simulink model "sf_fitness"  (R2025b)
settings: Solver=FixedStepAuto  StartTime=0.0  StopTime=inf  FixedStep=0.001  RelTol=1e-3  EnableMultiTasking=on
PreLoadFcn:
  | load sf_fitness_buses.mat;
StopFcn:
  | delete(app)
undefined symbols (not defined in the file or in its folder): ActivityType
CloseFcn:
  | clear app
  | clear FitnessDisplay
  | clear FitnessThresholds
  | clear FitnessVitals
settings Model: Creator=The MathWorks, Inc.  LastModifiedBy=The MathWorks, Inc.
settings SolverCC: AlgebraicLoopSolver=TrustRegion  IsAutoAppliedInSIP=on
settings DataIOCC: LimitDataPoints=on  SaveTime=off  ReturnWorkspaceOutputs=off
settings OptimizationCC: ReuseModelBlockBuffer=off  LifeSpan=inf
settings DebuggingCC: UnconnectedInputMsg=warning  UnconnectedOutputMsg=warning  UnconnectedLineMsg=warning  AllowSymbolicDim=off  PregeneratedLibrarySubsystemCodeDiagnostic=none  SFUnexpectedBacktrackingDiag=warning  SFNoUnconditionalDefaultTransitionDiag=warning  SFExecutionAtInitializationDiag=none  ArithmeticOperatorsInVariantConditions=warning
settings ModelReferenceCC: EnableRefExpFcnMdlSchedulingChecks=on  PropagateSignalLabelsOutOfModel=off
settings SFSimCC: SimUseLocalCustomCode=off  CustomCodeUndefinedFunction=UseInterfaceOnly
settings RTWCC: RTWUseLocalCustomCode=off  GPUComputeCapability=3.5  DLArmComputeVersion=19.05
settings CodeAppCC: StateflowObjectComments=on
settings GRTTargetCC: TargetLangStandard=C89/C90 (ANSI)
settings ConfigComp: CovMetricSettings=dw  CovSaveCumulativeToWorkspaceVar=on  CovSaveSingleToWorkspaceVar=on  CovExternalEMLEnable=off
settings SimscapeCC: SimscapeNormalizeSystem=off  SimscapeNominalValues={1, 'bar'; 1, 'cm^3/s'; 1, 'bar*kg/s'; 1, 'kJ/kg'; 1, 'kW'}

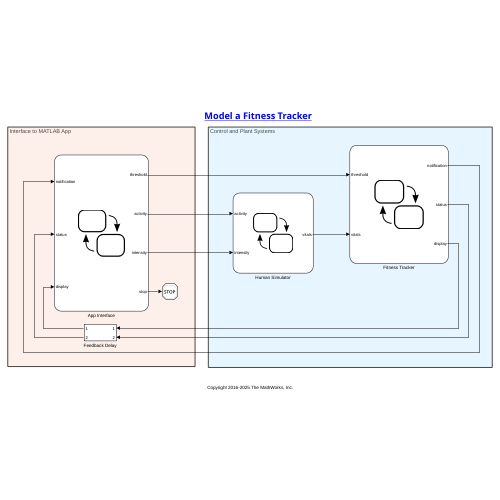
[thumbnail: Simulink's stored preview of the top-level diagram]
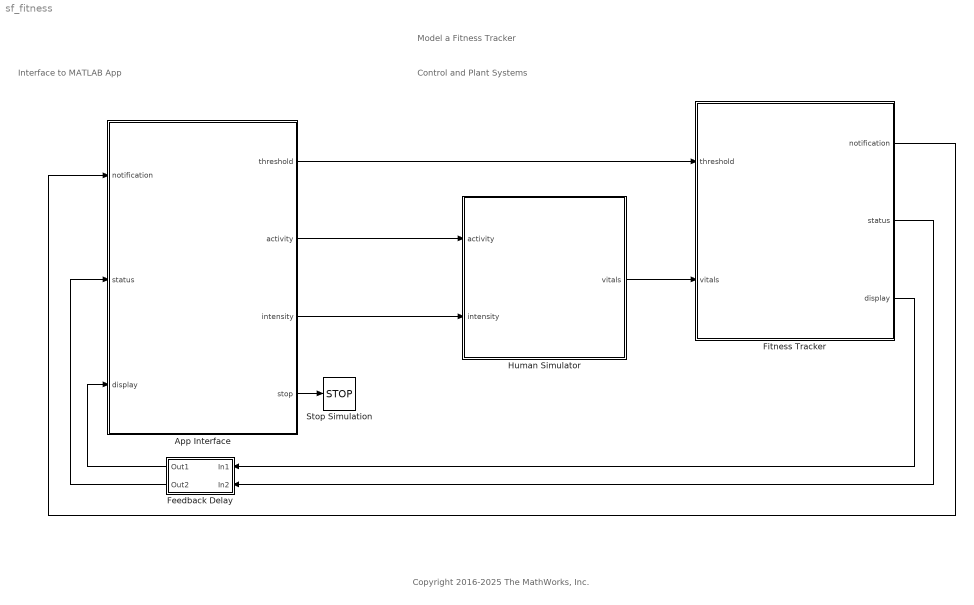
== system sf_fitness ==
  note: Control and Plant Systems
  note: Interface to MATLAB App
  note: Copyright 2016-2025 The MathWorks, Inc.
  note: Model a Fitness Tracker
  App Interface : Stateflow chart  TreatAsAtomicUnit=on
  Feedback Delay : Subsystem
  Fitness Tracker : Stateflow chart  TreatAsAtomicUnit=on
      settings: PortSchema="{\"entries\":[{\"content\":{\"sides\":[{\"content\":{\"connectorIds\":[\"In1\",\"In2\"]},\"type\":\"ConnectorPlacement.EquallySpacedRectSide\",\"uuid\":\"afd40bc3-205b-45f1-b484-c4f33cea0ca8\"},{\"content\":{\"connectorIds\":[\"Out1\",\"Out3\",\"Out2\"],\"side\":\"RIGHT\"},\"type\":\"ConnectorPlacement.EquallySpacedRectSide\",\"uuid\":\"d6f91233-35c5-46a8-af22-1c26ecf92787\"},{\"content\":{\"connectorIds\":[],\"side\":\"TOP\"},\"type\":\"ConnectorPlacement.EquallySpacedRectSide\",\"uuid\":\"b785bd09-019e-4ae9-a457-04601cbf60c7\"},{\"content\":{\"connectorIds\":[],\"side\":\"HIDDEN\"},\"type\":\"ConnectorPlacement.EquallySpacedRectSide\",\"uuid\":\"2c22bb70-70b2-4576-b4f3-3c6d9d9d65de\"}]},\"type\":\"ConnectorPlacement.EquallySpacedConnector\",\"uuid\":\"fb400832-b5be-41c1-a3a6-f64440305270\"}],\"packageUris\":[\"http://schema.mathworks.com/mf0/Connector/R2020b\"],\"version\":\"1.0\"}"
  Human Simulator : Stateflow chart  TreatAsAtomicUnit=on
  Stop Simulation : Stop
  wires:
  App Interface/4(stop) -> Stop Simulation/1
  App Interface/2(activity) -> Human Simulator/1(activity)
  App Interface/3(intensity) -> Human Simulator/2(intensity)
  Fitness Tracker/1(notification) -> App Interface/1(notification)
  Fitness Tracker/2(display) -> Feedback Delay/1(In1)
  Feedback Delay/2(Out2) -> App Interface/2(status)
  Feedback Delay/1(Out1) -> App Interface/3(display)
  App Interface/1(threshold) -> Fitness Tracker/1(threshold)
  Human Simulator/1(vitals) -> Fitness Tracker/2(vitals)
  Fitness Tracker/3(" status") -> Feedback Delay/2(In2)

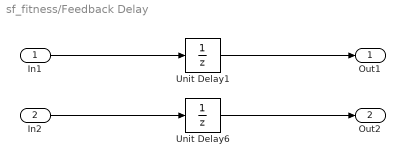
== system sf_fitness/Feedback Delay ==
  In1 : Inport
  In2 : Inport  Port=2
  Unit Delay1 : UnitDelay  SampleTime=-1  HasFrameUpgradeWarning=on
  Unit Delay6 : UnitDelay  InitialCondition=ActivityType.Rest  SampleTime=-1  HasFrameUpgradeWarning=on
  Out1 : Outport
  Out2 : Outport  Port=2
  wires:
  Unit Delay6/1 -> Out2/1
  In1/1 -> Unit Delay1/1
  Unit Delay1/1 -> Out1/1
  In2/1 -> Unit Delay6/1

== stateflow chart sf_fitness/Human Simulator ==
  note: Units for variables:
      | speed: number of steps per second
      | heart_rate: beats per minute
  state Simulator [parallel]
    en:
    vitals.heart_rate = 75;
    vitals.speed = 0;
    settings: executionOrder=1
    state Sim_Sleep
      en:
      oldhr = vitals.heart_rate;
      olds = vitals.speed;
      oldt = t;
      du:
      [vitals.heart_rate,vitals.speed] = sim_sleep(oldhr,olds,t-oldt);
    state Sim_Rest
      en:
      oldhr = vitals.heart_rate;
      olds = vitals.speed;
      oldt = t;
      du:
      [vitals.heart_rate,vitals.speed] = sim_rest(oldhr,olds,t-oldt);
    state Sim_Walk
      en:
      oldhr = vitals.heart_rate;
      olds = vitals.speed;
      oldt = t;
      du:
      [vitals.heart_rate,vitals.speed] = sim_walk(oldhr,olds,t-oldt);
    state Sim_Exercise
      en:
      oldhr = vitals.heart_rate;
      olds = vitals.speed;
      oldt = t;
      du:
      [vitals.heart_rate,vitals.speed] = sim_exercise(oldhr,olds,t-oldt,intensity);
    (default) -> (junction 353)
    (junction 353) -> (junction 257)
    (junction 257) -> Sim_Sleep [order 1] : [activity == ActivityType.Sleep]
    Sim_Sleep -> (junction 280)
    (junction 288) -> (junction 353)
    (junction 257) -> (junction 262) [order 2]
    (junction 280) -> (junction 281)
    (junction 262) -> Sim_Rest [order 1] : [activity == ActivityType.Rest]
    Sim_Rest -> (junction 281)
    (junction 262) -> (junction 264) [order 2]
    (junction 281) -> (junction 282)
    (junction 264) -> Sim_Walk [order 1] : [activity == ActivityType.Walk]
    Sim_Walk -> (junction 282)
    (junction 264) -> (junction 266) [order 2]
    (junction 282) -> (junction 286)
    (junction 266) -> Sim_Exercise : %[activity == ActivityType.Exercise]
    Sim_Exercise -> (junction 286)
    (junction 286) -> (junction 287)
    (junction 287) -> (junction 288) : [hasChanged(activity) || hasChanged(intensity)]
  state Step_Tracker [parallel]
    en: vitals.steps = 0;
    settings: executionOrder=2
    state Step
    (default) -> Step
    Step -> Step : after(1,sec){vitals.steps = vitals.steps + vitals.speed * 60;}
  data: oldHR function_input; oldS function_input; newTime function_input; heartRate function_output; Speed function_output; oldHR function_input; oldS function_input; newTime function_input; heartRate function_output; Speed function_output; oldHR function_input; oldS function_input; newTime function_input; heartRate function_output; Speed function_output; heartRate function_output; Speed function_output; oldHR function_input; oldS function_input; newTime function_input; Strength function_input; old function_input; target function_input; result function_output; t function_input; activity input Enum: ActivityType; intensity input; oldhr local; olds local; oldt local; vitals output Bus: FitnessVitals size=1
  function [heartRate, Speed] = sim_sleep(oldHR, oldS, newTime):
    | function [heartRate, Speed] = sim_sleep(oldHR, oldS, newTime)
    |    
    | target = 68;
    | 
    | % call transition function from oldHR to target
    | heartRate = transition(oldHR, target, newTime);
    | % update exercising speed
    | Speed = transition(oldS, 0, newTime);
    |     
    | end
  function [heartRate, Speed] = sim_rest(oldHR, oldS, newTime):
    | function [heartRate, Speed] = sim_rest(oldHR, oldS, newTime)
    |    
    | target = 75;
    | 
    | % call transition function from oldHR to target
    | heartRate = transition(oldHR, target, newTime);
    | % update exercising speed
    | Speed = transition(oldS, 0, newTime);
    |     
    | end
  function [heartRate, Speed] = sim_walk(oldHR, oldS, newTime):
    | function [heartRate, Speed] = sim_walk(oldHR, oldS, newTime)
    |    
    | target = 85;
    | 
    | % call transition function from oldHR to target
    | heartRate = transition(oldHR, target, newTime);
    | % update exercising speed
    | Speed = transition(oldS, 2, newTime);
    |     
    | end
  function [heartRate, Speed] = sim_exercise(oldHR, oldS, newTime, Strength):
    | function [heartRate, Speed] = sim_exercise(oldHR, oldS, newTime, Strength)
    | 
    | % strength is exercise level 1- 10
    | target = 85 + Strength * 8;
    | 
    | % call transition function from oldHR to target
    | heartRate = transition(oldHR, target, newTime);
    | % update exercising speed
    | % assume walk speed is 5
    | Speed = transition(oldS, (2 + 0.5 * Strength), newTime);
    | 
    | end
  function result = transition(old, target, t):
    | function result = transition(old, target, t)
    |     
    |     % use linear transition
    |     if t < 1 % all transition finish in 1 s; improve this later
    |         result = old + t * (target - old);
    |     else
    |         result = target;
    |     end
    |     
    | end

== stateflow chart sf_fitness/Fitness Tracker ==
  state TrackActivity
    display.heart_rate = vitals.heart_rate;
    display.total_steps = vitals.steps;
    state Rest
      exit:
      display.steps = 0;
      display.timer = elapsed(sec);
      state Need_Exercise [parallel]
        settings: executionOrder=1
        state Quiet
        state Notify
          en:
          notification.data = sf_fitness_NotificationType.Need_Exercise;
          send(notification);
        (default) -> TrackActivity.Rest.Need_Exercise.Quiet
        TrackActivity.Rest.Need_Exercise.Quiet -> TrackActivity.Rest.Need_Exercise.Notify : after(threshold.rest,sec)
      state Track_Steps [parallel]
        settings: executionOrder=2
        state Still
        state Moving
          en:
          init_steps = vitals.steps;
        (default) -> Still
        Still -> Moving : [vitals.speed > 0]
        Moving -> Still : [vitals.speed <= 0]
    state Exercise
      exit:
      display.steps = vitals.steps - init_steps;
      display.timer = elapsed(sec);
      state Timer [parallel]
        settings: executionOrder=1
        state Quiet
        state Notify
          en:
          notification.data = sf_fitness_NotificationType.Need_Rest;
          send(notification);
        (default) -> TrackActivity.Exercise.Timer.Quiet
        TrackActivity.Exercise.Timer.Quiet -> TrackActivity.Exercise.Timer.Notify : after(threshold.exercise,sec)
      state Exercise_Level [parallel]
        settings: executionOrder=2
        state Light_Exercise
        state Athlete
          state Init
          state Send
            en:
            notification.data = sf_fitness_NotificationType.Slow_Down;
            send(notification);
          (default) -> Init
          Init -> Send : after(15,sec)
        state Overheat
          en:
          notification.data = sf_fitness_NotificationType.Must_Stop;
          send(notification);
        (default) -> Light_Exercise
        Athlete -> Overheat [order 1] : [duration(vitals.heart_rate > threshold.heart_rate) > 1]
        Light_Exercise -> Athlete : [vitals.speed > 4]
        Athlete -> Light_Exercise [order 2] : [vitals.speed < 4]
        Overheat -> Athlete : [vitals.heart_rate < threshold.heart_rate]
      state Track_Steps [parallel]
        settings: executionOrder=3
        state Fast
        state Slow
          en:
          init_steps = vitals.steps;
        (default) -> Fast
        Fast -> Slow : [vitals.speed <= walk_speed]
        Slow -> Fast : [vitals.speed > walk_speed]
    state Walk
      exit:
      display.steps = vitals.steps - init_steps;
      display.timer = elapsed(sec);
      state Quiet
      state Notify
        ex:
        notification.data = sf_fitness_NotificationType.Report_Steps;
        send(notification);
      (default) -> TrackActivity.Walk.Quiet
      TrackActivity.Walk.Quiet -> TrackActivity.Walk.Notify : after(5,sec)
    state Sleep
      exit:
      display.steps = 0;
      display.timer = elapsed(sec);
      state Quiet
      state Notify
        ex:
        notification.data = sf_fitness_NotificationType.Sleep_Len;
        send(notification);
      (default) -> TrackActivity.Sleep.Quiet
      TrackActivity.Sleep.Quiet -> TrackActivity.Sleep.Notify : after(5,sec)
    (default) -> Rest
    (junction 320) -> Rest [order 1] : [vitals.speed == 0]
    Exercise -> (junction 320) : [duration(vitals.speed <= walk_speed) > 2]
    (junction 320) -> (junction 317) [order 2]
    Rest -> (junction 481) [order 2] : [duration(vitals.heart_rate <= sleep_heart_rate) > 2]
    (junction 481) -> Sleep
    Rest -> (junction 317) [order 1] : [duration(vitals.speed > 0) > 2]
    (junction 317) -> Exercise [order 1] : [vitals.speed > walk_speed]
    (junction 317) -> Walk [order 2]
    (junction 483) -> Rest
    (junction 486) -> Rest
    (junction 488) -> Exercise
    Walk -> (junction 486) [order 1] : [duration(vitals.speed == 0) > 2]
    Walk -> (junction 488) [order 2] : [duration(vitals.speed > walk_speed) > 2]
    Sleep -> (junction 483) : [duration(vitals.heart_rate >= rest_heart_rate) > 2]
  data: threshold input Bus: FitnessThresholds; notification output Enum: sf_fitness_NotificationType; sleep_heart_rate constant double =68; rest_heart_rate constant double =75; walk_speed constant double =2; init_steps local double size=1 =0; vitals input Bus: FitnessVitals; display output Bus: FitnessDisplay; status output Enum: ActivityType

== stateflow chart sf_fitness/App Interface ==
  state InterfaceWithApp
    en:
    coder.extrinsic('sf_fitness_app','updateStatus','updateClock','updateText','updateSteps','updateHeartRate');
    app = sf_fitness_app(this);
    initializeData();
    du:
    moving = detectMotion();
    interval = 30/display.heart_rate;
    state initializeData [function]
      (default) -> (junction 145) : {
          |  threshold.rest = 30;
          |  threshold.exercise = 40;
          |  threshold.heart_rate = 150;
          |  activity = ActivityType.Rest;
          |  intensity = 1;
          |  stop = false;
          | }
    state tf = detectMotion [function]
      (default) -> (junction 153)
      (junction 153) -> (junction 155) [order 1] : [status == ActivityType.Walk]
      (junction 153) -> (junction 159) [order 2]
      (junction 155) -> (junction 157)
      (junction 159) -> (junction 157) [order 1] : [status == ActivityType.Exercise]
      (junction 159) -> (junction 163) [order 2] : {tf = false;}
      (junction 157) -> (junction 165) : {tf = true;}
      (junction 163) -> (junction 165)
      (junction 165) -> (junction 168)
    state MainDisplay [parallel]
      % Clock and notifications
      settings: executionOrder=1
      state Clock
        en: updateClock(app,t);
      state Notification
        en: updateText(app,notification.data,t);
      (default) -> Clock
      Clock -> Notification [order 2] : notification
      Clock -> Clock [order 1] : after(1, sec)
      Notification -> Clock : after(5, sec)
    state Status [parallel]
      % New activity
      settings: executionOrder=2
      state Update
        en: updateStatus(app);
      (default) -> InterfaceWithApp.Status.Update
      InterfaceWithApp.Status.Update -> InterfaceWithApp.Status.Update : [hasChanged(status)]
    state Steps [parallel]
      % Total number of steps
      % and stepping animation
      settings: executionOrder=3
      state Silent
      state Update
        ex: updateSteps(app)
      (default) -> Silent
      Silent -> InterfaceWithApp.Steps.Update : [moving]
      InterfaceWithApp.Steps.Update -> Silent [order 1] : [~moving]
      InterfaceWithApp.Steps.Update -> InterfaceWithApp.Steps.Update [order 2] : after(0.5,sec)
    state HeartRate [parallel]
      % Heart rate and
      % heartbeat animation
      settings: executionOrder=4
      state Update
        en: updateHeartRate(app);
      (default) -> InterfaceWithApp.HeartRate.Update
      InterfaceWithApp.HeartRate.Update -> InterfaceWithApp.HeartRate.Update : after(interval,sec)
  data: tf function_output; threshold output Bus: FitnessThresholds; notification input; status input; interval local double; app local; activity output Enum: ActivityType; intensity output; stop output boolean; moving local boolean; display input Bus: FitnessDisplay
